simulink model "hover_plant_sil"  (R2025b)
settings: Solver=ode5  StartTime=0.0  StopTime=1  FixedStep=0.0000625  RelTol=1e-3
model workspace (MAT data in the model file):
  A = [0  0  0  1  0  0  0  0  0  0  0  0; 0  0  0  0  1  0  0  0  0  0  0  0; 0  0  0  0  0  1  0  0  0  0  0  0; 0  0  0  -1.35429089868  0  0  0  -9.81  0  0  0  0; 0  0  0  0  -1.35429089868  0  9.81  0  0  0  0  0; 0  0  0  0  0  -0.948003629075  0  0  0  0  0  0; 0  0  0  0  0  0  0  0  0  1  0  0; 0  0  0  0  0  0  0  0  0  0  1  0; 0  0  0  0  0  0  0  0  0  0  0  1; 0  0  0  0  0  0  0  0  0  -0.408828310259  0  0; 0  0  0  0  0  0  0  0  0  0  -0.406731754822  0; 0  0  0  0  0  0  0  0  0  0  0  -0.209821937011]
  Aomega = 0.486439179934
  Aref = 0.486439179934
  Ax = 0.243219589967
  Ay = 0.243219589967
  Az = 0.170253712977
  B = [0  0  0  0; 0  0  0  0; 0  0  0  0; 0  0  0  0; 0  0  0  0; -0.00416363636364  -0.00416363636364  -0.00416363636364  -0.00416363636364; 0  0  0  0; 0  0  0  0; 0  0  0  0; 0  -0.0259690721649  0  0.0259690721649; 0.0258358974359  0  -0.0258358974359  0; 0  0  0  0]
  C = [0  0  0  -1.35429089868  0  0  0  0  0  0  0  0; 0  0  0  0  -1.35429089868  0  0  0  0  0  0  0; 0  0  0  0  0  -0.948003629075  0  0  0  0  0  0; 0  0  0  0  0  0  0  0  0  1  0  0; 0  0  0  0  0  0  0  0  0  0  1  0; 0  0  0  0  0  0  0  0  0  0  0  1]
  C11 = 0.000458
  C21 = -0.562
  CDw = 1
  CDx = 1
  CDy = 1
  CDz = 1
  D = [0  0  0  0; 0  0  0  0; -0.00416363636364  -0.00416363636364  -0.00416363636364  -0.00416363636364; 0  0  0  0; 0  0  0  0; 0  0  0  0]
  I = [0.00194  0  0; 0  0.00195  0; 0  0  0.00378]
  Ix = 0.00194
  Iy = 0.00195
  Iz = 0.00378
  Lp = 0.000793126921902
  MMA = [1  0  1  1; 1  -1  0  -1; 1  0  -1  1; 1  1  0  -1]
  Mq = 0.000793126921902
  Nr = 0.000793126921902
  S = 0.11
  Ts = 0.00025
  X0 = [0; 0; 0; 0; 0; 0; 0; 0; 0; 0; 0; 0]
  Xref = [0; 0; 0; 0; 0; 0; 0; 0; 0; 0; 0; 0]
  Xu = 0.148971998855
  Yv = 0.148971998855
  Zw = 0.104280399198
  accel.range = 4
  accel.resolution_bits = 16
  accel.BW = 740
  accel.LPF_set = 5
  accel.sample_rate = 1600
  accel.noise_density = 0.00016
  accel.bias = [0.02; 0.02; 0.02]
  accel.vibration = 0.1
  accel.resolution_LSB = 0.000598754882813
  accel.alpha = 0.00779277730415
  accel.tau = 0.000215074247421
  bfConfig.Format = 'BetaflightSimulationConfig'
  bfConfig.SchemaVersion = 1
  bfConfig.CLI : char (value not decoded)
  bfConfig.SchemaText : char (value not decoded)
  bfConfig.Firmware.Repository = 'https://github.com/betaflight/betaflight'
  bfConfig.Firmware.Commit = 'c78d9e7bd24ef60f4324dffde11df26c53d4f29f'
  bfConfig.Firmware.Target = 'SITL'
  bfConfig.Firmware.Version = '2026.12.0-alpha'
  bfConfig.Firmware.HostProtocol = 1
  bfConfig.Firmware.GyroRateHz = 4000
  bfConfig.Firmware.Compiler = 'Cygwin GCC 13.5.0'
  bfRc = [1500; 1500; 1859; 1500; 1900; 1900; 1000; 1000; 1000; 1000; 1000; 1000; 1000; 1000; 1000; 1000]
  bfSim.SampleTime = 0.00025
  bfSim.TrimPot = 1816.10262009
  bfSim.InitialState = [0; 0; 0; 0; 0; 0; 0; 0; 0; 0; 0; 0]
  bfSim.WarmupSeconds = 5
  bfSim.ArmSettleSeconds = 0.3
  bfSim.SpoolupSeconds = 1
  bfSim.Timeout = 5
  bfSim.NavigationSensors = 0
  bfSim.RcRateHz = 100
  bfSim.UseKnownAccelCalibration = 1
  bfSim.CommandMode = 'angle'
  bfSim.ThrottlePWM = 1859
  bfSim.MotorOrder = [1 2 3 4]
  bfSim.TraceFile = ''
  bfSim.ReceiverPWM = []
  bfSim.StartupReceiverPWM = []
  bfSim.ReferenceSchedule = []
  bfSim.ReceiverLayout.Roll = 1
  bfSim.ReceiverLayout.Pitch = 2
  bfSim.ReceiverLayout.Throttle = 3
  bfSim.ReceiverLayout.Yaw = 4
  bfSim.ReceiverLayout.Arm = 5
  bfSim.ReceiverLayout.ArmOn = 1900
  bfSim.ReceiverLayout.ArmOff = 1000
  bfSim.ReceiverLayout.Angle = 6
  bfSim.ReceiverLayout.AngleOn = 1900
  bfSim.ReceiverLayout.AngleOff = 1000
  bfSim.ReceiverLayout.Ranges = [1000  2000; 1000  2000; 1000  2000; 1000  2000]
  bfSim.ReceiverLayout.MidRc = 1500
  bfSim.CalibrationGyro = [0.00872664625997; 0.00872664625997; 0.00872664625997]
  bfSim.CalibrationAccelBias = [0.1962; 0.1962; 0.1962]
  bfSim.CalibrationGyroNoiseStd = 0.189395809295
  bfSim.CalibrationGyroSampleTime = 0.0003125
  bfSim.CalibrationSeed = 23341
  bfSim.Gravity = 9.81
  bfSim.PidSampleTime = 0.00025
  bfSim.MinThrottlePWM = 1000
  drag_enabled = 1
  fs = 4000
  g = 9.81
  gyro.range = 1000
  gyro.resolution_bits = 16
  gyro.BW = 751
  gyro.LPF_set = 5
  gyro.sample_rate = 3200
  gyro.noise_density = 0.007
  gyro.bias = [0.5; 0.5; 0.5]
  gyro.vibration = 3.7
  gyro.resolution_LSB = 0.000532632218016
  gyro.alpha = 0.00779277730415
  gyro.tau = 0.000211924025422
  imu_nonlinear = 1
  k_tau = 0
  m = 0.11
  mahoney.Kp = 0.25
  mahoney.Ki = 0.05
  max_pot = 1950
  noise_true = 1
  p_ref = 1
  pitch_D = 0
  pitch_I = 0.00502577319588
  pitch_P = 0.0221134020619
  q_ref = 1
  r_ref = 1
  rho = 1.225
  roll_D = 0
  roll_I = 0.005
  roll_P = 0.022
  seed = 23341
  sil_accel_noise_power = [0.0018230966784; 0.0018230966784; 0.0018230966784]
  sil_gyro_noise_power = [1.12096164307e-05; 1.12096164307e-05; 1.12096164307e-05]
  sim_fidelity = 'high'
  strength = 50
  t_sim = 10
  tau_p = 0.2
  tau_q = 0.2
  tau_r = 0.4
  tau_wing = 0.0454545454545
  u0 = 1816.10262009
  use_time_constant_damping = 0
  v_ref = 0.5
  w_ref = 0.5
  wing_area = 0.121609794983
  wing_type = 15
  yaw_D = 0
  yaw_I = 0.001
  yaw_P = 0.001
  yaw_row = [0 0 0 0]
undefined symbols (not defined in the file): dspblkCoreblockFVToolHelper, gcbh
libraries: simulink x3, simulink_extras x1
settings Model: Creator=bmatt  LastModifiedBy=bmatt
settings DataIOCC: SignalLogging=off
settings OptimizationCC: EnhancedBackFolding=on  PassReuseOutputArgsAs=Individual arguments  ZeroExternalMemoryAtStartup=off  ZeroInternalMemoryAtStartup=off  OptimizeBlockOrder=speed  DifferentSizesBufferReuse=on  OptimizationCustomize=off  EfficientTunableParamExpr=on
settings DebuggingCC: ParameterTunabilityLossMsg=error
settings SFSimCC: MATLABDynamicMemAlloc=off
settings RTWCC: SystemTargetFile=ert.tlc  GenCodeOnly=on  TemplateMakefile=ert_default_tmf  Description=Embedded Coder
settings CodeAppCC: ForceParamTrailComments=on  IgnoreCustomStorageClasses=off  OperatorAnnotations=on  SimulinkDataObjDesc=on  SFDataObjDesc=on  CustomSymbolStrUtil=hover_plant_sil_$N$C  InsertBlockDesc=on
settings ERTTargetCC: InlinedParameterPlacement=Hierarchical  ERTCustomFileTemplate=example_file_process.tlc  TargetLangStandard=C99 (ISO)  CombineOutputUpdateFcns=off  SupportContinuousTime=on

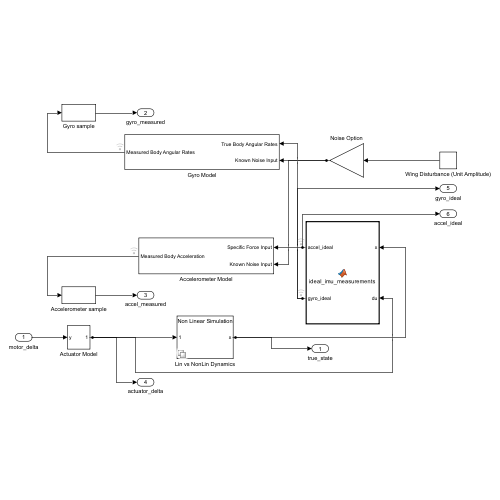
[thumbnail: Simulink's stored preview of the top-level diagram]
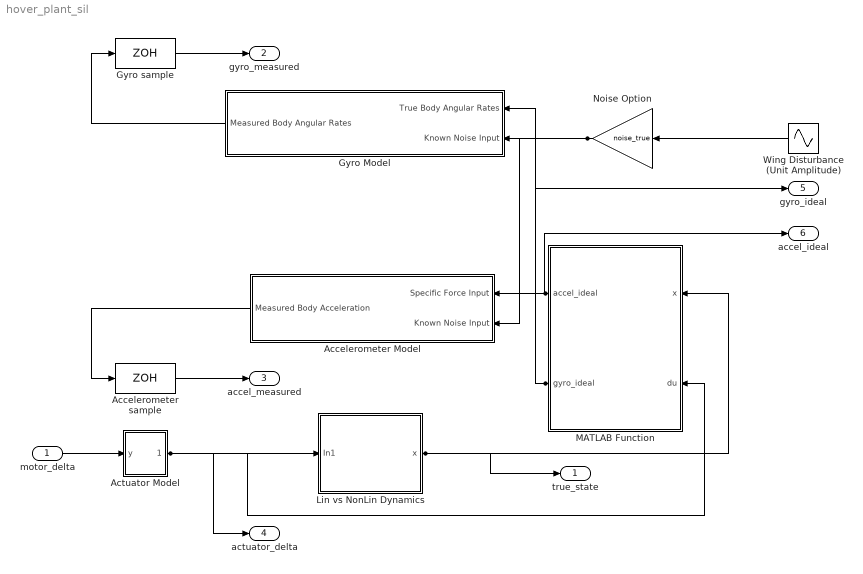
== system hover_plant_sil ==
  motor_delta : Inport  PortDimensions=4  SampleTime=Ts
  Accelerometer Model : Subsystem
  Accelerometer sample : ZeroOrderHold  SampleTime=Ts
  Actuator Model : Subsystem
  Gyro Model : Subsystem
  Gyro sample : ZeroOrderHold  SampleTime=Ts
  Lin vs NonLin Dynamics : Subsystem  Variant=on
  MATLAB Function : MATLAB Function  TreatAsAtomicUnit=on
  Noise Option : Gain  Gain=noise_true
  Wing Disturbance (Unit Amplitude) : Sin  Frequency=2*pi*24  SampleTime=0
  true_state : Outport
  gyro_measured : Outport  Port=2
  accel_measured : Outport  Port=3
  actuator_delta : Outport  Port=4
  gyro_ideal : Outport  Port=5
  accel_ideal : Outport  Port=6
  wires:
  motor_delta/1 -> Actuator Model/1(y)
  Noise Option/1 -> Accelerometer Model/2(Known Noise Input), Gyro Model/2(Known Noise Input)
  Accelerometer Model/1(Measured Body Acceleration) -> Accelerometer sample/1
  Gyro sample/1 -> gyro_measured/1
  Actuator Model/1(Out1) -> MATLAB Function/2(du), Lin vs NonLin Dynamics/1(In1), actuator_delta/1
  Accelerometer sample/1 -> accel_measured/1
  Gyro Model/1(Measured Body Angular Rates) -> Gyro sample/1
  Lin vs NonLin Dynamics/1(x) -> MATLAB Function/1(x), true_state/1
  MATLAB Function/2(gyro_ideal) -> Gyro Model/1(True Body Angular Rates), gyro_ideal/1
  MATLAB Function/1(accel_ideal) -> accel_ideal/1, Accelerometer Model/1(Specific Force Input)
  Wing Disturbance (Unit Amplitude)/1 -> Noise Option/1

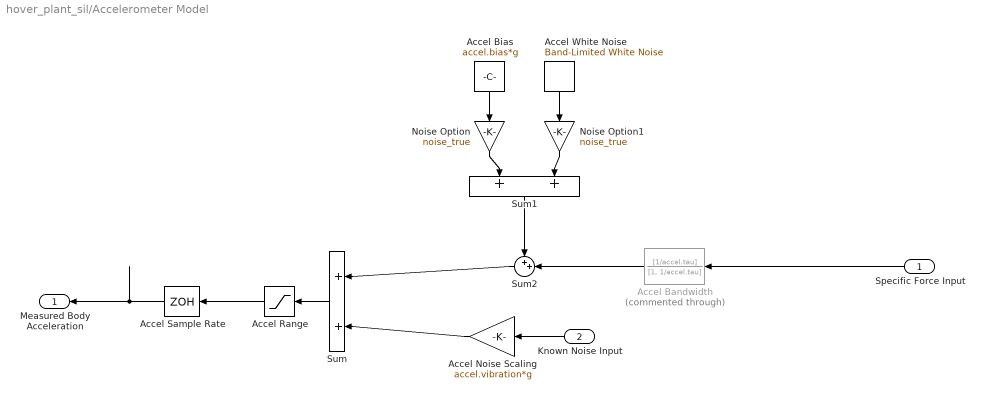
== system hover_plant_sil/Accelerometer Model ==
  Specific Force Input : Inport
  Known Noise Input : Inport  Port=2
  Accel White Noise : simulink/Sources/Band-Limited White Noise  Cov=sil_accel_noise_power  Ts=1/accel.sample_rate  seed=[seed]
  Accel Bandwidth : DiscreteTransferFcn  Commented=through  LoadFcn=dspblkCoreblockFVToolHelper(gcbh,'load');  Numerator=[1/accel.tau]  Denominator=[1, 1/accel.tau]
      settings: CopyFcn=dspblkCoreblockFVToolHelper(gcbh,'copy');  DeleteFcn=dspblkCoreblockFVToolHelper(gcbh,'close');  ModelCloseFcn=dspblkCoreblockFVToolHelper(gcbh,'close');  PreSaveFcn=dspblkCoreblockFVToolHelper(gcbh,'presave');  PostSaveFcn=dspblkCoreblockFVToolHelper(gcbh,'postsave');  CloseFcn=dspblkCoreblockFVToolHelper(gcbh,'close');
  Accel Bias : Constant  Value=accel.bias*g  SampleTime=1/accel.sample_rate
  Accel Noise Scaling : Gain  Gain=accel.vibration*g
  Accel Range : Saturate  UpperLimit=4*9.81  LowerLimit=-4*9.81
  Accel Sample Rate : ZeroOrderHold  SampleTime=1/accel.sample_rate
  Noise Option : Gain  Gain=noise_true
  Noise Option1 : Gain  Gain=noise_true
  Sum : Sum  Inputs=+|+
  Sum1 : Sum  Inputs=+|+
  Sum2 : Sum  Inputs=++|
  Measured Body Acceleration : Outport
  wires:
  Accel White Noise/1 -> Noise Option1/1
  Noise Option1/1 -> Sum1/2
  Accel Bias/1 -> Noise Option/1
  Noise Option/1 -> Sum1/1
  Accel Range/1 -> Accel Sample Rate/1
  Accel Noise Scaling/1 -> Sum/2
  Sum1/1 -> Sum2/1
  Specific Force Input/1 -> Accel Bandwidth/1
  Accel Bandwidth/1 -> Sum2/2
  Known Noise Input/1 -> Accel Noise Scaling/1
  Accel Sample Rate/1 -> Measured Body Acceleration/1
  Sum2/1 -> Sum/1
  Sum/1 -> Accel Range/1

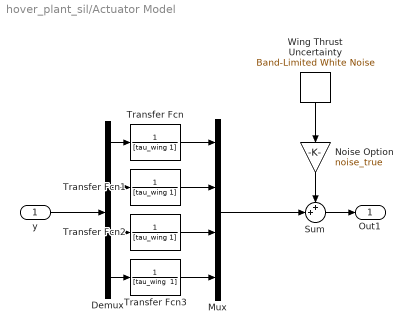
== system hover_plant_sil/Actuator Model ==
  y : Inport
  Demux : Demux
  Mux : Mux
  Noise Option : Gain  Gain=noise_true
  Sum : Sum  Inputs=++|
  Transfer Fcn : TransferFcn  Denominator=[tau_wing 1]
  Transfer Fcn1 : TransferFcn  Denominator=[tau_wing 1]
  Transfer Fcn2 : TransferFcn  Denominator=[tau_wing 1]
  Transfer Fcn3 : TransferFcn  Denominator="[tau_wing  1]"
  Wing Thrust Uncertainty : simulink/Sources/Band-Limited White Noise  Cov=1*[0.000001566122567;0.000001566122567;0.000001566122567;0.000001566122567]  Ts=Ts  seed=[seed]
  Out1 : Outport
  wires:
  Noise Option/1 -> Sum/1
  Wing Thrust Uncertainty/1 -> Noise Option/1
  Mux/1 -> Sum/2
  Sum/1 -> Out1/1
  y/1 -> Demux/1
  Transfer Fcn3/1 -> Mux/4
  Transfer Fcn2/1 -> Mux/3
  Transfer Fcn1/1 -> Mux/2
  Transfer Fcn/1 -> Mux/1
  Demux/3 -> Transfer Fcn2/1
  Demux/2 -> Transfer Fcn1/1
  Demux/1 -> Transfer Fcn/1
  Demux/4 -> Transfer Fcn3/1

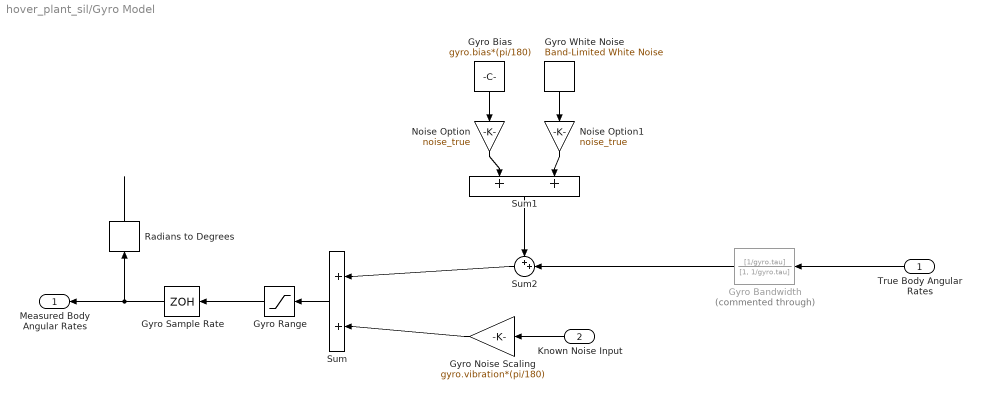
== system hover_plant_sil/Gyro Model ==
  True Body Angular Rates : Inport
  Known Noise Input : Inport  Port=2
  Gyro White Noise : simulink/Sources/Band-Limited White Noise  Cov=sil_gyro_noise_power  Ts=1/gyro.sample_rate  seed=[seed]
  Gyro Bandwidth : DiscreteTransferFcn  Commented=through  LoadFcn=dspblkCoreblockFVToolHelper(gcbh,'load');  Numerator=[1/gyro.tau]  Denominator=[1, 1/gyro.tau]
      settings: CopyFcn=dspblkCoreblockFVToolHelper(gcbh,'copy');  DeleteFcn=dspblkCoreblockFVToolHelper(gcbh,'close');  ModelCloseFcn=dspblkCoreblockFVToolHelper(gcbh,'close');  PreSaveFcn=dspblkCoreblockFVToolHelper(gcbh,'presave');  PostSaveFcn=dspblkCoreblockFVToolHelper(gcbh,'postsave');  CloseFcn=dspblkCoreblockFVToolHelper(gcbh,'close');
  Gyro Bias : Constant  Value=gyro.bias*(pi/180)  SampleTime=1/gyro.sample_rate
  Gyro Noise Scaling : Gain  Gain=gyro.vibration*(pi/180)
  Gyro Range : Saturate  UpperLimit=1000*(pi/180)  LowerLimit=-1000*(pi/180)
  Gyro Sample Rate : ZeroOrderHold  SampleTime=1/gyro.sample_rate
  Noise Option : Gain  Gain=noise_true
  Noise Option1 : Gain  Gain=noise_true
  Radians to Degrees : simulink_extras/Transformations/Radians to Degrees
  Sum : Sum  Inputs=+|+
  Sum1 : Sum  Inputs=+|+
  Sum2 : Sum  Inputs=++|
  Measured Body Angular Rates : Outport
  wires:
  Radians to Degrees/1 -> ?
  Noise Option1/1 -> Sum1/2
  Gyro White Noise/1 -> Noise Option1/1
  Gyro Bias/1 -> Noise Option/1
  Noise Option/1 -> Sum1/1
  Gyro Noise Scaling/1 -> Sum/2
  Sum2/1 -> Sum/1
  Gyro Range/1 -> Gyro Sample Rate/1
  Gyro Sample Rate/1 -> Measured Body Angular Rates/1, Radians to Degrees/1
  Gyro Bandwidth/1 -> Sum2/2
  Sum1/1 -> Sum2/1
  Known Noise Input/1 -> Gyro Noise Scaling/1
  Sum/1 -> Gyro Range/1
  True Body Angular Rates/1 -> Gyro Bandwidth/1

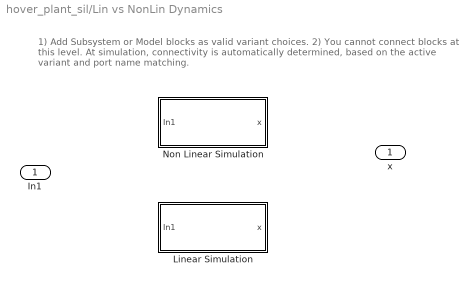
== system hover_plant_sil/Lin vs NonLin Dynamics ==
  note: 1) Add Subsystem or Model blocks as valid variant choices.
      | 2) You cannot connect blocks at this level. At simulation, connectivity is automatically
      | determined, based on the active variant and port name matching.
  In1 : Inport
  Linear Simulation : Subsystem  VariantControl=false
  Non Linear Simulation : Subsystem  VariantControl=true
  x : Outport

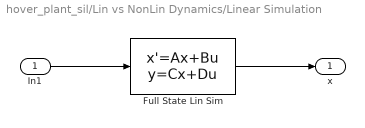
== system hover_plant_sil/Lin vs NonLin Dynamics/Linear Simulation ==
  In1 : Inport
  Full State Lin Sim : StateSpace  A=A  B=B  C=eye(12)  D=zeros(12,4)  InitialCondition=X0
  x : Outport
  wires:
  Full State Lin Sim/1 -> x/1
  In1/1 -> Full State Lin Sim/1

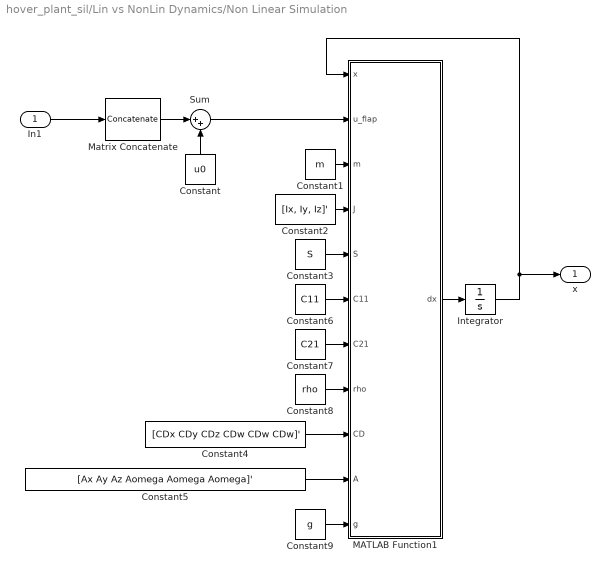
== system hover_plant_sil/Lin vs NonLin Dynamics/Non Linear Simulation ==
  In1 : Inport
  Constant : Constant  Value=u0
  Constant1 : Constant  Value=m
  Constant2 : Constant  Value=[Ix, Iy, Iz]'
  Constant3 : Constant  Value=S
  Constant4 : Constant  Value=[CDx CDy CDz CDw CDw CDw]'
  Constant5 : Constant  Value=[Ax Ay Az Aomega Aomega Aomega]'
  Constant6 : Constant  Value=C11
  Constant7 : Constant  Value=C21
  Constant8 : Constant  Value=rho
  Constant9 : Constant  Value=g
  Integrator : Integrator  InitialCondition=X0
  MATLAB Function1 : MATLAB Function  TreatAsAtomicUnit=on
  Matrix Concatenate : Concatenate  NumInputs=1
  Sum : Sum  Inputs=|++
  x : Outport
  wires:
  Matrix Concatenate/1 -> Sum/1
  Constant9/1 -> MATLAB Function1/11(g)
  Constant4/1 -> MATLAB Function1/9(CD)
  Constant6/1 -> MATLAB Function1/6(C11)
  Constant8/1 -> MATLAB Function1/8(rho)
  Constant7/1 -> MATLAB Function1/7(C21)
  Constant5/1 -> MATLAB Function1/10(A)
  Constant3/1 -> MATLAB Function1/5(S)
  Constant2/1 -> MATLAB Function1/4(J)
  Constant1/1 -> MATLAB Function1/3(m)
  Constant/1 -> Sum/2
  Sum/1 -> MATLAB Function1/2(u_flap)
  In1/1 -> Matrix Concatenate/1
  Integrator/1 -> x/1, MATLAB Function1/1(x)
  MATLAB Function1/1(dx) -> Integrator/1

== matlab function hover_plant_sil/MATLAB Function ==
  data: x input; accel_ideal output; du input; gyro_ideal output; m parameter; g parameter; C11 parameter; Xu parameter; Yv parameter; Zw parameter; rho parameter; CDx parameter; CDy parameter; CDz parameter; Ax parameter; Ay parameter; Az parameter; imu_nonlinear parameter
function [accel_ideal,gyro_ideal]=ideal_imu_measurements(x,du,m,g,C11,Xu,Yv,Zw,rho,CDx,CDy,CDz,Ax,Ay,Az,imu_nonlinear)
%#codegen
[accel_ideal,gyro_ideal]=bf.idealImu(x,du,m,g,C11,[Xu;Yv;Zw], ...
    0.5*rho*[CDx*Ax;CDy*Ay;CDz*Az],imu_nonlinear);
end

== matlab function hover_plant_sil/Lin vs NonLin Dynamics/Non Linear Simulation/MATLAB Function1 ==
  data: x input; dx output size=12; u_flap input; m input; J input; S input; C11 input; C21 input; rho input; CD input; A input; g input
function dx = nonlinearEOM(x,u_flap,m,J,S,C11,C21,rho,CD,A,g)
%#codegen
% x      = [x y z u v w phi theta psi p q r]'
% u_flap = absolute flapper commands [u1 u2 u3 u4]' [pot]
% J      = [Ix Iy Iz]'
% CD     = [CDx CDy CDz CDp CDq CDr]'
% A      = [Ax Ay Az Ap Aq Ar]'
% Body/inertial z positive down; 3-2-1 Euler angles

u=x(4); v=x(5); w=x(6); ph=x(7); th=x(8); ps=x(9);
p=x(10); q=x(11); r=x(12); Ix=J(1); Iy=J(2); Iz=J(3);

% Actual flapper thrusts, positive upward (-z body)
T = C11*u_flap + C21;

% Quadratic translational drag + total flapper thrust
F = -.5*rho*CD(1:3).*A(1:3).*abs([u;v;w]).*[u;v;w];
F(3) = F(3) - sum(T);

% Flapper moments + quadratic rotational drag
M = [S*(T(4)-T(2)); S*(T(1)-T(3)); 0] ...
    - .5*rho*CD(4:6).*A(4:6)*S^3.*abs([p;q;r]).*[p;q;r];

% Nonlinear translational dynamics
vd = F/m + [-g*sin(th); g*sin(ph)*cos(th); g*cos(ph)*cos(th)] ...
     - cross([p;q;r],[u;v;w]);

% Nonlinear rotational dynamics
wd = [(M(1)-(Iz-Iy)*q*r)/Ix;
      (M(2)-(Ix-Iz)*p*r)/Iy;
      (M(3)-(Iy-Ix)*p*q)/Iz];

% Exact 3-2-1 Euler-angle kinematics
E = [1 sin(ph)*tan(th) cos(ph)*tan(th);
     0 cos(ph)        -sin(ph);
     0 sin(ph)/cos(th) cos(ph)/cos(th)];

% Inertial-to-body DCM
C_bI = [cos(th)*cos(ps), cos(th)*sin(ps), -sin(th);
        sin(ph)*sin(th)*cos(ps)-cos(ph)*sin(ps), ...
        sin(ph)*sin(th)*sin(ps)+cos(ph)*cos(ps), sin(ph)*cos(th);
        cos(ph)*sin(th)*cos(ps)+sin(ph)*sin(ps), ...
        cos(ph)*sin(th)*sin(ps)-sin(ph)*cos(ps), cos(ph)*cos(th)];

% Full state derivative
dx = [C_bI'*[u;v;w]; vd; E*[p;q;r]; wd];
end
